simulink model "FBL_simulation"  (R2025a)
settings: Solver=ode4  StartTime=0.0  StopTime=200  FixedStep=0.001  RelTol=1e-3
undefined symbols (not defined in the file or in its folder): p
settings Model: Creator=Giammo  LastModifiedBy=Giammo
settings SolverCC: ZeroCrossAlgorithm=Adaptive
settings DebuggingCC: IgnoredZcDiagnostic=none

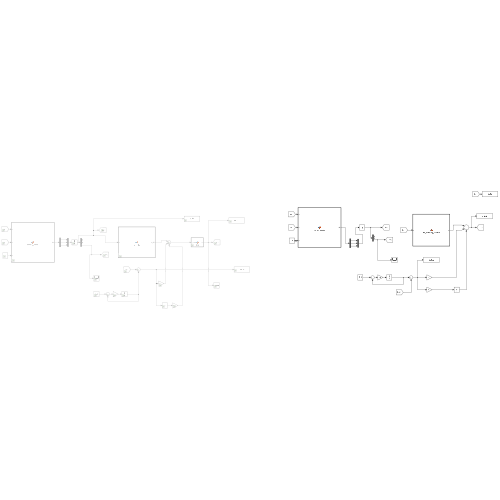
[thumbnail: Simulink's stored preview of the top-level diagram]
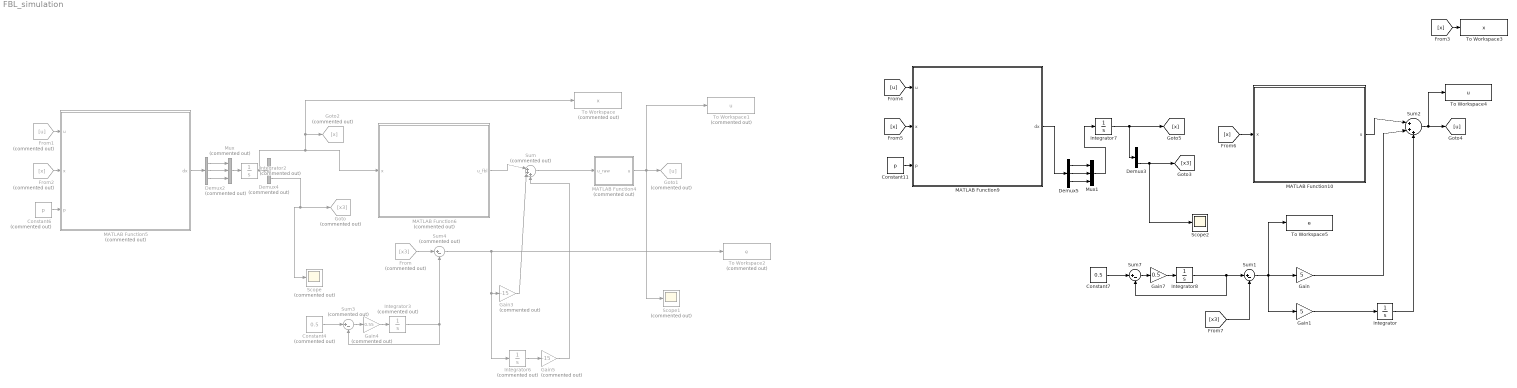
== system FBL_simulation ==
  Constant11 : Constant  Value=p  OutDataTypeStr=Bus: slBus1
  Constant4 : Constant  Commented=on  Value=0.5
  Constant6 : Constant  Commented=on  Value=p  OutDataTypeStr=Bus: slBus1
  Constant7 : Constant  Value=0.5
  Demux2 : Demux  Commented=on  Outputs=3
  Demux3 : Demux  Outputs=3
  Demux4 : Demux  Commented=on  Outputs=3
  Demux5 : Demux  Outputs=3
  From : From  Commented=on  GotoTag=x3
  From1 : From  Commented=on  GotoTag=u
  From2 : From  Commented=on  GotoTag=x
  Gain : Gain  Gain=5
  Gain1 : Gain  Gain=5
  Gain3 : Gain  Commented=on  Gain=-15
  Gain4 : Gain  Commented=on  Gain=0.55
  Gain5 : Gain  Commented=on  Gain=-15
  Gain7 : Gain  Gain=0.5
  Goto : Goto  Commented=on  GotoTag=x3
  Goto1 : Goto  Commented=on  GotoTag=u
  Goto2 : Goto  Commented=on  GotoTag=x
  Integrator : Integrator  InitialCondition=0.4
  Integrator2 : Integrator  Commented=on  InitialCondition=[0.1;0.1;0.1]  LowerSaturationLimit=[0;0;0]
  Integrator3 : Integrator  Commented=on  InitialCondition=0.4
  Integrator6 : Integrator  Commented=on  InitialCondition=0.4  LowerSaturationLimit=-1
  Integrator7 : Integrator  InitialCondition=[0.9;0.1;0.1]  LowerSaturationLimit=[0;0;0]
  Integrator8 : Integrator
  MATLAB Function10 : MATLAB Function  TreatAsAtomicUnit=on
  MATLAB Function4 : MATLAB Function  Commented=on  TreatAsAtomicUnit=on
  MATLAB Function5 : MATLAB Function  Commented=on  TreatAsAtomicUnit=on
  MATLAB Function6 : MATLAB Function  Commented=on  TreatAsAtomicUnit=on
  MATLAB Function9 : MATLAB Function  TreatAsAtomicUnit=on
  Mux : Mux  Commented=on  Inputs=3
  Mux1 : Mux  Inputs=3
  Scope : Scope  Commented=on
      settings: ActiveDisplayYMinimum=-0.012491096495775927  ActiveDisplayYMaximum=1.1124198684619837
  Scope1 : Scope  Commented=on
      settings: ActiveDisplayYMinimum=-0.010599435528881686  ActiveDisplayYMaximum=0.29937018747967792
  Scope2 : Scope
      settings: ActiveDisplayYMinimum=0.031071942826426224  ActiveDisplayYMaximum=0.66092327783020632  DataLoggingVariableName=ScopeData2
  Sum : Sum  Commented=on  Inputs=|+++
  Sum1 : Sum  Inputs=|+-
  Sum2 : Sum  Inputs=|+++
  Sum3 : Sum  Commented=on  Inputs=|+-
  Sum4 : Sum  Commented=on  Inputs=|+-
  Sum7 : Sum  Inputs=|+-
  To Workspace : ToWorkspace  Commented=on  VariableName=x  SaveFormat=Timeseries  SampleTime=-1
  To Workspace1 : ToWorkspace  Commented=on  VariableName=u  SaveFormat=Timeseries  SampleTime=-1
  To Workspace2 : ToWorkspace  Commented=on  VariableName=e  SaveFormat=Timeseries  SampleTime=-1
  To Workspace3 : ToWorkspace  VariableName=x  SaveFormat=Timeseries  SampleTime=-1
  To Workspace4 : ToWorkspace  VariableName=u  SaveFormat=Timeseries  SampleTime=-1
  To Workspace5 : ToWorkspace  VariableName=e  SaveFormat=Timeseries  SampleTime=-1
  wires:
  Constant6/1 -> MATLAB Function5/3(p)
  Sum3/1 -> Gain4/1
  Gain4/1 -> Integrator3/1
  MATLAB Function6/1(u_fbl) -> Sum/1
  From/1 -> Sum4/1
  Sum4/1 -> Gain3/1, Integrator6/1, To Workspace2/1
  Gain3/1 -> Sum/2
  From1/1 -> MATLAB Function5/1(u)
  From2/1 -> MATLAB Function5/2(x)
  Integrator3/1 -> Sum3/2, Sum4/2
  Integrator6/1 -> Gain5/1
  Gain5/1 -> Sum/3
  MATLAB Function4/1(u) -> Scope1/1, Goto1/1, To Workspace1/1
  Sum/1 -> MATLAB Function4/1(u_raw)
  [u] -> MATLAB Function9/1(u)
  Sum7/1 -> Gain7/1
  Integrator7/1 -> [x], Demux3/1
  Integrator8/1 -> Sum1/1, Sum7/2
  Constant11/1 -> MATLAB Function9/3(p)
  [x] -> MATLAB Function9/2(x)
  Gain7/1 -> Integrator8/1
  Constant7/1 -> Sum7/1
  Constant4/1 -> Sum3/1
  MATLAB Function5/1(dx) -> Demux2/1
  Demux2/1 -> Mux/1
  Demux2/2 -> Mux/2
  Mux/1 -> Integrator2/1
  Integrator2/1 -> To Workspace/1, Goto2/1, MATLAB Function6/1(x), Demux4/1
  Demux4/3 -> Goto/1, Scope/1
  Demux5/2 -> Mux1/2
  Demux5/1 -> Mux1/1
  Mux1/1 -> Integrator7/1
  MATLAB Function9/1(dx) -> Demux5/1
  Demux3/3 -> Scope2/1, [x3]
  Demux5/3 -> Mux1/3
  [x] -> To Workspace3/1
  [x] -> MATLAB Function10/1(x)
  [x3] -> Sum1/2
  Sum1/1 -> To Workspace5/1, Gain1/1, Gain/1
  MATLAB Function10/1(u) -> Sum2/1
  Gain/1 -> Sum2/2
  Gain1/1 -> Integrator/1
  Integrator/1 -> Sum2/3
  Sum2/1 -> To Workspace4/1, [u]
  Demux2/3 -> Mux/3

== matlab function FBL_simulation/MATLAB Function4 ==
  data: u_raw input; u output
function u = fcn(u_raw)
    % Map the raw command smoothly to a value between zero and one.
    
    u = 1 / (1 + exp(-u_raw)); 
end

== matlab function FBL_simulation/MATLAB Function5 ==
  data: u input; dx output; x input; p input
function dx = cancer_model(u, x, p)
    % Continuous-time dynamics: states are tumor, hunting cells and resting cells; u acts on x3.

    x1 = x(1);
    x2 = x(2);
    x3 = x(3);
    A12 = p.A12;
    A13 = p.A13;
    R2  = p.R2;
    A21 = p.A21;
    R3  = p.R3;
    k3  = p.k3;
    A31 = p.A31;
    D3  = p.D3;
    dx = zeros(3,1);
    dx(1) = x1*(1 - x1) - A12*x1*x2 - A13*x1*x3;
    dx(2) = R2*x2*(1 - x2) - A21*x1*x2;
    recruitment = (R3 * x1 * x3) / (x1 + k3);
    dx(3) = recruitment - A31*x1*x3 - D3*x3 + u;

end

== matlab function FBL_simulation/MATLAB Function6 ==
  data: x input; u_fbl output
function u_fbl = IO_FBL(x)
    % Cancel the resting-cell drift for the output y = x3, whose input gain is one.
   
    R2 = 0.6; R3 = 4.5; D3 = 0.5;
    A12 = 1.0; A21 = 1.5; A13 = 2.5; A31 = 0.2; k3 = 1;
    x1 = x(1); 
    x2 = x(2); 
    x3 = x(3); 
    Lf_h = (R3*x1*x3)/(x1 + k3) - A31*x1*x3 - D3*x3;
    Lg_h = 1; 
    u_fbl = (-Lf_h) / 1;
end

== matlab function FBL_simulation/MATLAB Function10 ==
  data: x input; u output
function u  = fbl_switching_control(x)
    % Split the drift-canceling command into bounded stimulation and inhibition.
   
    R2 = 0.6; R3 = 4.5; D3 = 0.5;
    A12 = 1.0; A21 = 1.5; A13 = 2.5; A31 = 0.2; k3 = 1;
    u_max_stim = 1.0;  
    u_max_inh  = -1.0; 
    f3_x = (R3 * x(1) * x(3)) / (x(1) + k3) - A31 * x(1) * x(3) - D3 * x(3);
    u_ideal = -f3_x ;
    if u_ideal >= 0
        u_stim  = min(u_ideal, u_max_stim);
        u_inhib = 0;                        
    else
        u_stim  = 0;                        
        u_inhib = max(u_ideal, u_max_inh);  
    end
    u = u_stim + u_inhib;
    
end

== matlab function FBL_simulation/MATLAB Function9 ==
  data: u input; dx output; x input; p input
function dx = cancer_model(u, x, p)
    % Continuous-time dynamics: states are tumor, hunting cells and resting cells; u acts on x3.

    x1 = x(1);
    x2 = x(2);
    x3 = x(3);
    A12 = p.A12;
    A13 = p.A13;
    R2  = p.R2;
    A21 = p.A21;
    R3  = p.R3;
    k3  = p.k3;
    A31 = p.A31;
    D3  = p.D3;
    dx = zeros(3,1);
    dx(1) = x1*(1 - x1) - A12*x1*x2 - A13*x1*x3;
    dx(2) = R2*x2*(1 - x2) - A21*x1*x2;
    recruitment = (R3 * x1 * x3) / (x1 + k3);
    dx(3) = recruitment - A31*x1*x3 - D3*x3 + u;

end
